simulink model "limo"  (R2023b)
settings: Solver=FixedStepAuto  StartTime=0.0  StopTime=10  FixedStep=1e-5  RelTol=1e-3
values from neighbouring files (symbols this model uses):
  k_alpha = 20    [fichierlimo.m]
  k_beta = -10    [fichierlimo.m]
  k_rho = 1    [fichierlimo.m]
  L = 322e-3    (= 0.322)    [fichierlimo.m]
  theta0 = 0    [fichierlimo.m]
  theta_star = 0    [fichierlimo.m]
  x0 = 0.5    [fichierlimo.m]
  x_star = -0.5    [fichierlimo.m]
  y0 = 1    [fichierlimo.m]
  y_star = 2    [fichierlimo.m]
settings Model: Creator=sabri  LastModifiedBy=MissVava

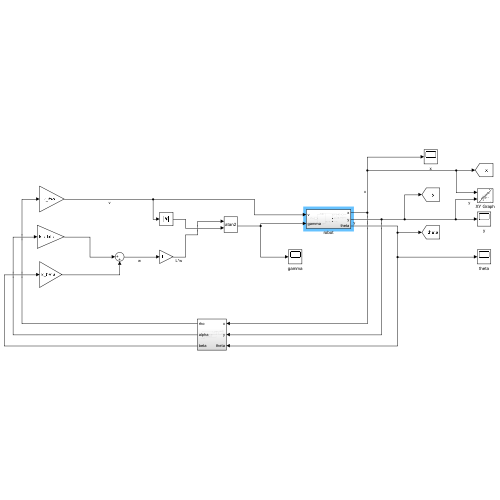
[thumbnail: Simulink's stored preview of the top-level diagram]
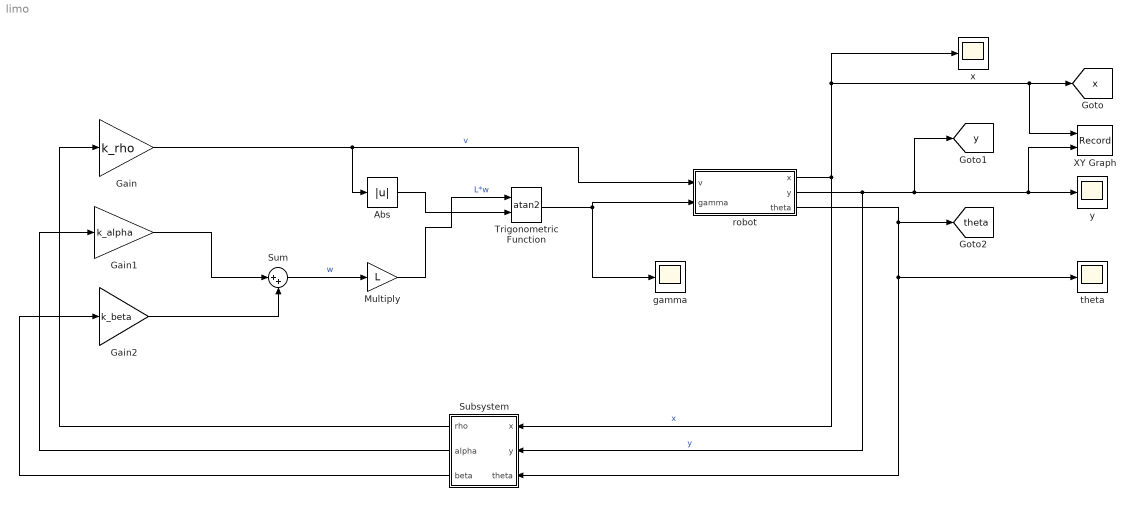
== system limo ==
  Abs : Abs  SaturateOnIntegerOverflow=off
  Gain : Gain  Gain=k_rho
  Gain1 : Gain  Gain=k_alpha
  Gain2 : Gain  Gain=k_beta
  Multiply : Gain  Gain=L
  Subsystem : Subsystem
  Sum : Sum  Inputs=|++
  Trigonometric Function : Trigonometry  Operator=atan2
  XY Graph : Record  FileSettingsInternal="{\"entries\":[{\"content\":{\"excelSettings\":{\"content\":{},\"type\":\"Streamout.ExcelSettings\"}},\"type\":\"Streamout.FileSettingStorage\",\"uuid\":\"\"}],\"packageUris\":[\"http:\\/\\/schema.mathworks.com\\/mf0\\/streamout_blocks\\/R2020a\"],\"version\":\"1.0\"}"  Layout=[1 1]  SignalsInternal="{\"entries\":[{\"content\":{\"signals\":[{\"content\":{\"blockPath\":[],\"dimensions\":[1],\"domain\":\"\",\"lineColor\":\"#a2142f\",\"plots\":[1],\"port\":1,\"sid\":[\"\"],\"signalID\":4567,\"signalName\":\"x\"},\"type\":\"RecordBlkView.Signal\",\"uuid\":\"\"},{\"content\":{\"blockPath\":[],\"dimensions\":[1],\"domain\":\"\",\"lineColor\":\"#139fff\",\"plots\":[1],\"port\":2,\"sid\":[\"\"],\"signalID\":4571,\"signalName\":\"y\"},\"type\":\"RecordBlkView.Signal\",\"uuid\":\"\"}]},\"type\":\"RecordBlkView.InputSignals\",\"uuid\":\"\"}],\"packageUris\":[\"http:\\/\\/schema.mathworks.com\\/mf0\\/streamout_blocks\\/R2020a\"],\"version\":\"1.0\"}"  VisualizationBindings="{\"xyplotplugin\":{\"info\":[{\"series\":[{\"bindingParametersList\":[{\"parameter\":\"X-Axis\",\"signalID\":4567,\"signalName\":\"x\"},{\"parameter\":\"Y-Axis\",\"signalID\":4571,\"signalName\":\"y\"}],\"seriesID\":30538}],\"subplotID\":1}]}}"  CompatibilityTag=XY
  gamma : Scope
  robot : Subsystem
  theta : Scope
  x : Scope
  y : Scope
  tag scope: theta=global, x=global, y=global
  wires:
  Gain1/1 -> Sum/1
  Gain2/1 -> Sum/2
  Sum/1 -> Multiply/1  "w"
  Gain/1 -> Abs/1, robot/1(v)  "v"
  robot/1(x) -> [x], XY Graph/1, x/1, Subsystem/1(x)  "x"
  robot/2(y) -> [y], XY Graph/2, y/1, Subsystem/2(y)  "y"
  robot/3(theta) -> Subsystem/3(theta), theta/1, [theta]
  Subsystem/1(rho) -> Gain/1
  Subsystem/2(alpha) -> Gain1/1
  Subsystem/3(beta) -> Gain2/1
  Trigonometric Function/1 -> robot/2(gamma), gamma/1
  Multiply/1 -> Trigonometric Function/1  "L*w"
  Abs/1 -> Trigonometric Function/2

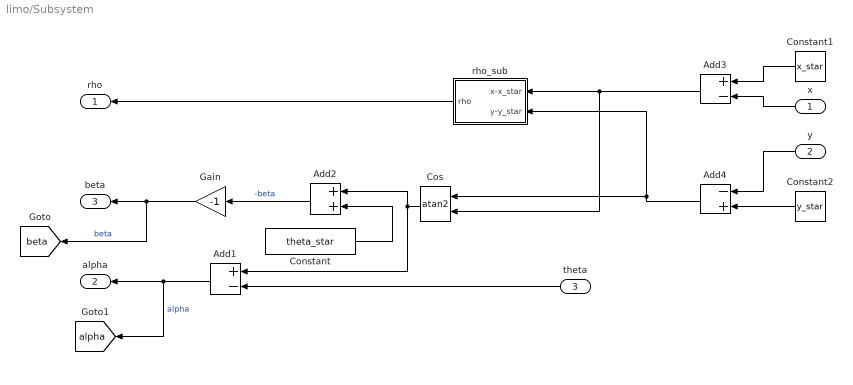
== system limo/Subsystem ==
  x : Inport
  y : Inport  Port=2
  theta : Inport  Port=3
  Add1 : Sum  Inputs=+-
  Add2 : Sum
  Add3 : Sum  Inputs=+-
  Add4 : Sum  Inputs=-+
  Constant : Constant  Value=theta_star
  Constant1 : Constant  Value=x_star
  Constant2 : Constant  Value=y_star
  Cos : Trigonometry  Operator=atan2
  Gain : Gain  Gain=-1
  rho_sub : Subsystem
  rho : Outport
  alpha : Outport  Port=2
  beta : Outport  Port=3
  tag scope: alpha=global, beta=global
  wires:
  Add4/1 -> Cos/1, rho_sub/2(y-y_star)
  rho_sub/1(rho) -> rho/1
  Gain/1 -> [beta], beta/1  "beta"
  Add2/1 -> Gain/1  "-beta"
  Constant/1 -> Add2/2
  Cos/1 -> Add2/1, Add1/1
  Add1/1 -> [alpha], alpha/1  "alpha"
  theta/1 -> Add1/2
  Constant2/1 -> Add4/2
  Constant1/1 -> Add3/1
  x/1 -> Add3/2
  y/1 -> Add4/1
  Add3/1 -> Cos/2, rho_sub/1(x-x_star)

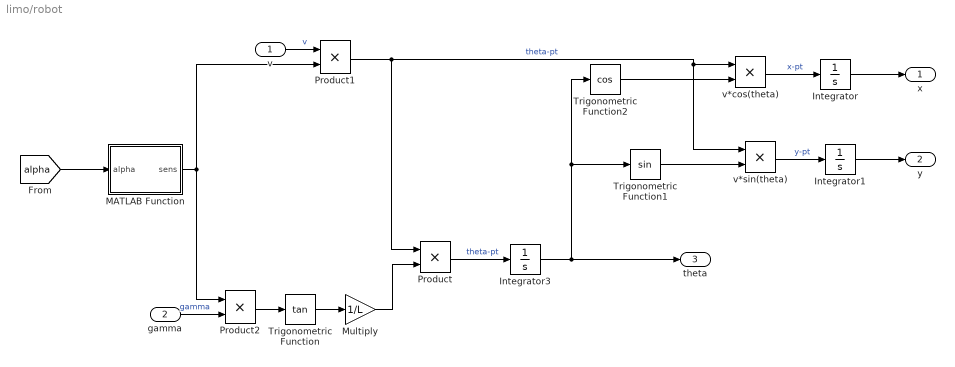
== system limo/robot ==
  v : Inport
  gamma : Inport  Port=2
  Integrator : Integrator  InitialCondition=x0
  Integrator1 : Integrator  InitialCondition=y0
  Integrator3 : Integrator  InitialCondition=theta0
  MATLAB Function : MATLAB Function  TreatAsAtomicUnit=on
  Multiply : Gain  Gain=1/L
  Product : Product
  Product1 : Product
  Product2 : Product
  Trigonometric Function : Trigonometry  Operator=tan
  Trigonometric Function1 : Trigonometry
  Trigonometric Function2 : Trigonometry  Operator=cos
  v*cos(theta) : Product
  v*sin(theta) : Product
  x : Outport
  y : Outport  Port=2
  theta : Outport  Port=3
  wires:
  Trigonometric Function/1 -> Multiply/1
  Product2/1 -> Trigonometric Function/1
  Multiply/1 -> Product/2
  Product/1 -> Integrator3/1  "theta-pt"
  Trigonometric Function2/1 -> v*cos(theta)/2
  v*cos(theta)/1 -> Integrator/1  "x-pt"
  v*sin(theta)/1 -> Integrator1/1  "y-pt"
  Trigonometric Function1/1 -> v*sin(theta)/2
  Integrator3/1 -> theta/1, Trigonometric Function2/1, Trigonometric Function1/1
  Integrator1/1 -> y/1
  Integrator/1 -> x/1
  MATLAB Function/1(sens) -> Product2/1, Product1/2
  v/1 -> Product1/1  "v"
  Product1/1 -> v*sin(theta)/1, v*cos(theta)/1, Product/1  "theta-pt"
  gamma/1 -> Product2/2  "gamma"
  [alpha] -> MATLAB Function/1(alpha)

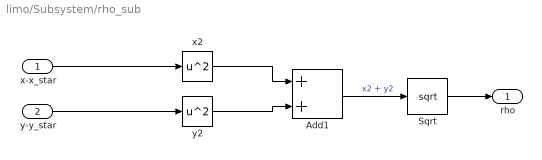
== system limo/Subsystem/rho_sub ==
  x-x_star : Inport
  y-y_star : Inport  Port=2
  Add1 : Sum
  Sqrt : Sqrt
  x2 : Math  Operator=square
  y2 : Math  Operator=square
  rho : Outport
  wires:
  x2/1 -> Add1/1
  y2/1 -> Add1/2
  Add1/1 -> Sqrt/1  "x2 + y2"
  Sqrt/1 -> rho/1
  x-x_star/1 -> x2/1
  y-y_star/1 -> y2/1

== matlab function limo/robot/MATLAB Function ==
  data: alpha input; sens output
function sens = fcn(alpha)
    if (alpha >= -1.57 && alpha <= 1.57)
        sens = 1;
    else
        sens = -1;
    end
end
